simulink model "InfusionPumpPlantModel"  (R2022b)
settings: Solver=ode23t  StartTime=0.0  StopTime=10.0  MaxStep=0.001  RelTol=1e-3
undefined symbols (not defined in the file): const_Occl_Pct, reserv_str
libraries: fl_lib x44, nesl_utility x21, sh_lib x7, sdl_lib x4, ee_lib x1, simulink_extras x1, fl_ps_legacy_lib x1
settings Model: Creator=szhang  LastModifiedBy=ppatel
settings SolverCC: AlgebraicLoopSolver=TrustRegion
settings DebuggingCC: UnconnectedInputMsg=warning  UnconnectedOutputMsg=warning  UnconnectedLineMsg=warning  SFMachineParentedDataDiag=warning  ArithmeticOperatorsInVariantConditions=warning
settings ModelReferenceCC: EnableRefExpFcnMdlSchedulingChecks=on
settings SFSimCC: SimUseLocalCustomCode=off  CustomCodeUndefinedFunction=UseInterfaceOnly
settings RTWCC: RTWUseLocalCustomCode=off
settings CodeAppCC: StateflowObjectComments=on
settings SimscapeCC: SimscapeNominalValues="[{\"value\":\"10\",\"unit\":\"V\"},{\"value\":\"1\",\"unit\":\"A\"},{\"value\":\"10\",\"unit\":\"N*m\"},{\"value\":\"10\",\"unit\":\"bar\"},{\"value\":\"100\",\"unit\":\"kJ/kg\"},{\"value\":\"1\",\"unit\":\"kW\"},{\"value\":\"300\",\"unit\":\"K\"},{\"value\":\"100\",\"unit\":\"cm^3/s\"},{\"value\":\"1\",\"unit\":\"kN\"},{\"value\":\"1\",\"unit\":\"g/cm^3\"},{\"value\":\"1\",\"unit\":\"l\"},{\"value\":\"1\",\"unit\":\"cm^2\"},{\"value\":\"60\",\"unit\":\"Hz\"}]"

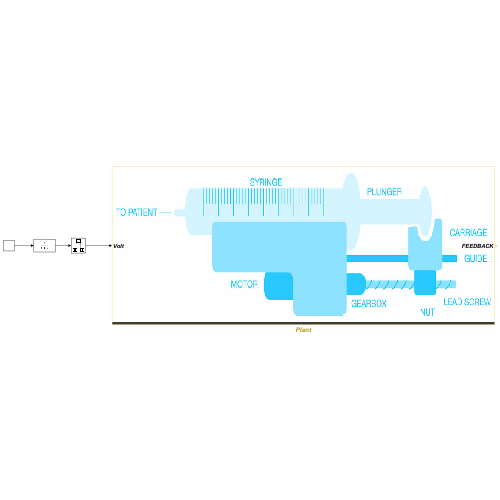
[thumbnail: Simulink's stored preview of the top-level diagram]
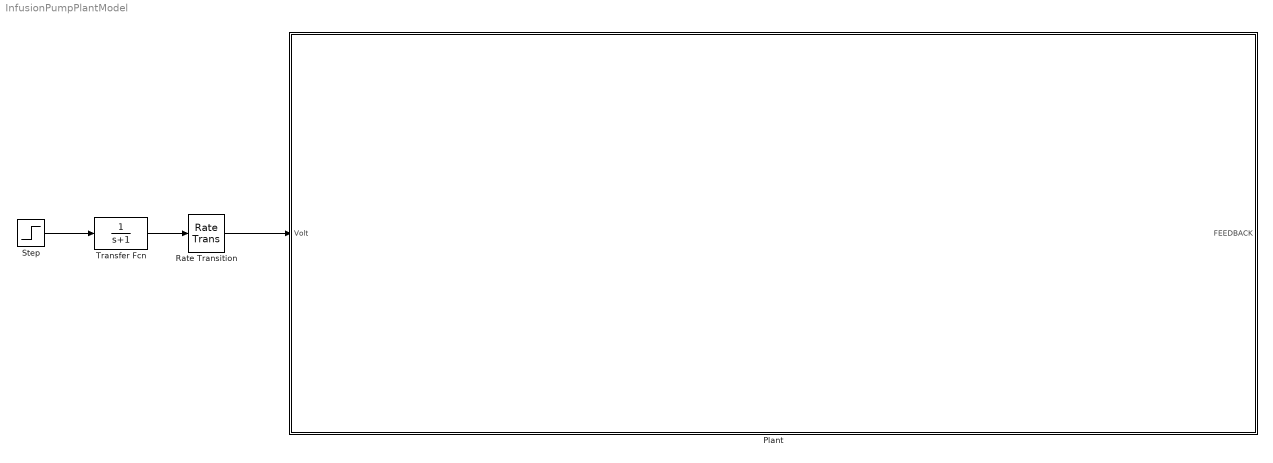
== system InfusionPumpPlantModel ==
  Plant : Subsystem
      mask Display: image('InfusionDevice.PNG');
  Rate Transition : RateTransition  OutPortSampleTime=0.001
  Step : Step  After=2.5  SampleTime=0
  Transfer Fcn : TransferFcn  Denominator=[1 1]
  wires:
  Rate Transition/1 -> Plant/1(Volt)
  Step/1 -> Transfer Fcn/1
  Transfer Fcn/1 -> Rate Transition/1

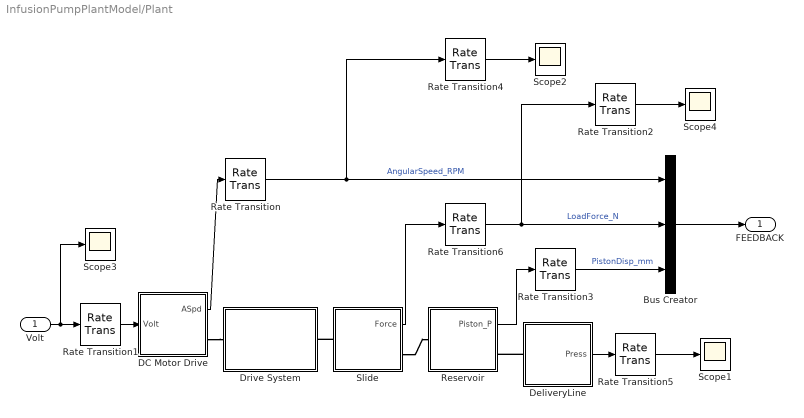
== system InfusionPumpPlantModel/Plant ==
  Volt : Inport
  Bus Creator : BusCreator  Inputs='AngularSpeed_RPM','LoadForce_N','PistonDisp_mm'  OutDataTypeStr=Bus: FEEDBACK  NonVirtualBus=on
  DC Motor Drive : Subsystem
      mask Display: image('DCMotor.PNG')
  DeliveryLine : Subsystem
      mask Display: image('DeliveryLine.PNG')
  Drive System : Subsystem
      mask Display: image('DriveSys.PNG')
  Rate Transition : RateTransition  OutPortSampleTime=0.001
  Rate Transition1 : RateTransition
  Rate Transition2 : RateTransition  OutPortSampleTime=0.01
  Rate Transition3 : RateTransition  OutPortSampleTime=0.001
  Rate Transition4 : RateTransition  OutPortSampleTime=0.01
  Rate Transition5 : RateTransition  OutPortSampleTime=0.01
  Rate Transition6 : RateTransition  OutPortSampleTime=0.001
  Reservoir : Subsystem
      mask Display: image('Reservoir.PNG')
  Scope{1..4} (4 alike) : Scope
  Slide : Subsystem
  FEEDBACK : Outport  OutDataTypeStr=Bus: FEEDBACK
  wires:
  DC Motor Drive/1(ASpd) -> Rate Transition/1
  Volt/1 -> Scope3/1, Rate Transition1/1
  Rate Transition1/1 -> DC Motor Drive/1(Volt)
  DeliveryLine/1(Press) -> Rate Transition5/1
  Rate Transition3/1 -> Bus Creator/3  "PistonDisp_mm"
  Reservoir/1(Piston_P) -> Rate Transition3/1
  Rate Transition/1 -> Rate Transition4/1, Bus Creator/1  "AngularSpeed_RPM"
  Rate Transition4/1 -> Scope2/1
  Rate Transition5/1 -> Scope1/1
  Slide/1(Force) -> Rate Transition6/1
  Rate Transition6/1 -> Rate Transition2/1, Bus Creator/2  "LoadForce_N"
  Bus Creator/1 -> FEEDBACK/1
  Rate Transition2/1 -> Scope4/1
  connections:
  Slide/RConn1 -- Reservoir/LConn1
  DC Motor Drive/RConn1 -- Drive System/LConn1
  Slide/LConn1 -- Drive System/RConn1
  DeliveryLine/LConn1 -- Reservoir/RConn1

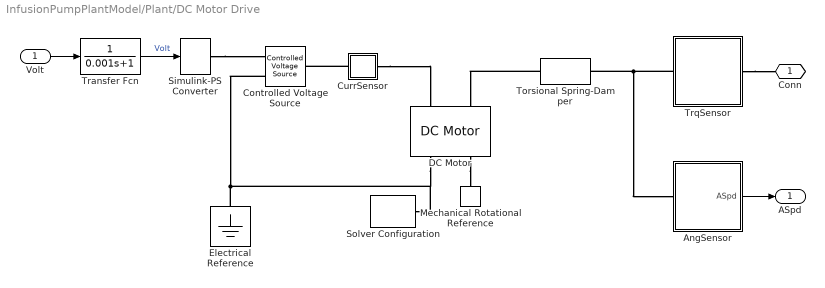
== system InfusionPumpPlantModel/Plant/DC Motor Drive ==
  Volt : Inport
  AngSensor : Subsystem
  Controlled Voltage Source : fl_lib/Electrical/Electrical Sources/Controlled Voltage Source
  CurrSensor : Subsystem
  DC Motor : ee_lib/Electromechanical/Brushed Motors/DC Motor  field_option=ee.enum.field_option.pm  Rf=100 Ohm  Lf=1 H  Laf=0.15 H  If0=0 A  parameterization=1  Ra=reserv_str.DCMotor.Resist Ohm  La=reserv_str.DCMotor.Induct H  emf_or_torque=1  Kv=reserv_str.DCMotor.BEMF V/(rad/s)  Ki=6.876e-4 N*m/A  T_stall=2.4e-4 N*m  w_max=1.91e+4 rpm  w_rated=1.5e+4 rpm  P_rated=0.08 W  V_rated=1.5 V  lam_param=1  i_noload=0 A  V_i_noload=1.5 V  J=reserv_str.DCMotor.RotorInert kg*m^2  lam=reserv_str.DCMotor.RotorDamp N*m/(rad/s)  speed0=0 rpm  enable_fault_armature=simscape.enum.onoff.off  rev_faulted=1 / 3  G_faulted_armature=1e-5 S  fault_trigger_armature=ee.enum.faults.faultTrigger.temporal  t_fault_armature=1 s  max_permissible_current_armature=inf A  t_fail_on_current_armature=1 s  enable_fault_field=simscape.enum.onoff.off  G_faulted_field=1e-5 S  fault_trigger_field=ee.enum.faults.faultTrigger.temporal  t_fault_field=1 s  max_permissible_current_field=inf A  t_fail_on_current_field=1 s  fault_action=simscape.enum.assert.action.none  alpha=3.93e-3 1/K  Tmeas=25 degC  thermal_mass=100 J/K  initial_temperature=25 degC
  Electrical Reference : fl_lib/Electrical/Electrical Elements/Electrical Reference
  Mechanical Rotational Reference : fl_lib/Mechanical/Rotational Elements/Mechanical Rotational Reference
  Simulink-PS Converter : nesl_utility/Simulink-PS Converter  PhysicalDomain=network_engine_domain  SubClassName=ps_input  LeftPortType=input  RightPortType=output  PseudoPeriodic=off  Frequencies=[]  NoiseDistribution=none  NoiseParameters=[]  Unit=1  AffineConversion=off  FilteringAndDerivatives=filter  SimscapeFilterOrder=2  InputFilterTimeConstant=0.001  UdotUserProvided=1
  Solver Configuration : nesl_utility/Solver Configuration  PhysicalDomain=network_engine_domain  SubClassName=solver  LeftPortType=input  RightPortType=generic  Tones=[]  Harmonics=[]  SimulateNoise=off  Profile=off  UseLocalSampling=off  EnableSwitchedLinearOptims=on  FrequencyDomain=off  UseCCode=off  RelTol=0.001  AbsTol=1e-06  MinStep=1e-09  ToWorkspace=off  RevertToSquareIcSolve=off  NumHomotopyIterations=100  PhasorMode=off  PhasorModeNumHarmonics=1  ConsistencySolver=NEWTON_XTOL_AFTER_FTOL  IndexReductionMethod=DerivativeReplacement  DoDC=off  ResidualTolerance=1e-09  ConsistencyTolSource=GLOBAL  ConsistencyAbsTol=0.001  ConsistencyRelTol=0.001  ConsistencyTolFactor=0.001  UseLocalSolver=off  LocalSolverChoice=NE_BACKWARD_EULER_ADVANCER  ResolveIndetEquations=on  FunctionEvalNumThread=1  LocalSolverSampleTime=0.001  DoFixedCost=off  MaxNonlinIter=3  MaxModeIter=2  ComputeImpulses=off  ImpulseIterations=2  LinearAlgebra=Sparse  LinearAlgebraNumThread=0  EquationFormulation=NE_TIME_EF  DelaysMemoryBudget=1024  AutomaticFiltering=on  FilteringTimeConstant=0.001  PartitionStorageMethod=AS_NEEDED  PartitionMemoryBudget=1024  PartitionMethod=FAST
  Torsional Spring-Damper : sdl_lib/Couplings & Drives/Torsional Spring-Damper  k=10000 N*m/rad  mu_visc=1000 N*m/(rad/s)  trq_coulomb=0 N*m  static_kinetic_ratio=1.1  w_tol=0.001 rad/s  model_hardstop=0  upper_bound=10 deg  lower_bound=-10 deg  k_endstop=1e+6 N*m/rad  D_endstop=10 N*m/(rad/s)  hardstop_model=3  transition=0.001 rad  x0=0 deg
      settings: InternalSimscapePortConfiguration="{\"Bottom\":[],\"Left\":[{\"id\":\"R\",\"label\":\"R\",\"type\":\"foundation.mechanical.rotational.rotational\"}],\"Right\":[{\"id\":\"C\",\"label\":\"C\",\"type\":\"foundation.mechanical.rotational.rotational\"}],\"Top\":[]}"
  Transfer Fcn : TransferFcn  Denominator=[0.001 1]
  TrqSensor : Subsystem
  Conn : PMIOPort  Side=Right
  ASpd : Outport
  wires:
  Volt/1 -> Transfer Fcn/1
  Transfer Fcn/1 -> Simulink-PS Converter/1  "Volt"
  AngSensor/1(ASpd) -> ASpd/1
  connections:
  Controlled Voltage Source/RConn2 -- Solver Configuration/RConn1 -- DC Motor/RConn1 -- Electrical Reference/LConn1
  DC Motor/RConn2 -- Mechanical Rotational Reference/LConn1
  Simulink-PS Converter/RConn1 -- Controlled Voltage Source/RConn1
  TrqSensor/RConn1 -- Conn/RConn1
  TrqSensor/LConn1 -- AngSensor/LConn1 -- Torsional Spring-Damper/RConn1
  CurrSensor/LConn1 -- Controlled Voltage Source/LConn1
  CurrSensor/RConn1 -- DC Motor/LConn1
  Torsional Spring-Damper/LConn1 -- DC Motor/LConn2

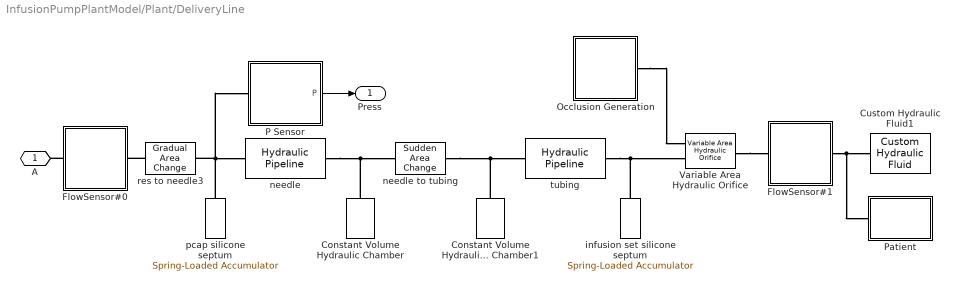
== system InfusionPumpPlantModel/Plant/DeliveryLine ==
  Constant Volume Hydraulic Chamber : fl_lib/Hydraulic/Hydraulic Elements/Constant Volume Hydraulic Chamber  ch_sp=1  wall_type=1  ch_volume=pi/4*reserv_str.Needle.Diam^2*reserv_str.Needle.Len/5 in^3  d_in=1e-2 m  length=1 m  pr_r_coef=1.2e-12 m/Pa  time_const=0.01 s  k_sh=1.4  pressure_specify=on  pressure_priority=High  pressure=reserv_str.Needle.InitP Pa  pressure_nominal_specify=off  pressure_nominal_unit=Pa  pressure_nominal_value=1  diameter_incr_specify=off  diameter_incr_priority=High  diameter_incr=0 m  diameter_incr_nominal_specify=off  diameter_incr_nominal_unit=m  diameter_incr_nominal_value=1  flow_rate_specify=off  flow_rate_priority=None  flow_rate=0.001 m^3/s  flow_rate_nominal_specify=off  flow_rate_nominal_unit=m^3/s  flow_rate_nominal_value=1
      settings: InternalSimscapePortConfiguration="{\"Bottom\":[],\"Left\":[{\"id\":\"A\",\"label\":\"\",\"type\":\"foundation.hydraulic.hydraulic\"}],\"Right\":[],\"Top\":[]}"
  Constant Volume Hydraulic Chamber1 : fl_lib/Hydraulic/Hydraulic Elements/Constant Volume Hydraulic Chamber  ch_sp=1  wall_type=1  ch_volume=pi/4*reserv_str.Tubing.Diam^2*reserv_str.Tubing.Len/5 in^3  d_in=1e-2 m  length=1 m  pr_r_coef=1.2e-12 m/Pa  time_const=0.01 s  k_sh=1.4  pressure_specify=on  pressure_priority=High  pressure=reserv_str.Needle.InitP Pa  pressure_nominal_specify=off  pressure_nominal_unit=Pa  pressure_nominal_value=1  diameter_incr_specify=off  diameter_incr_priority=High  diameter_incr=0 m  diameter_incr_nominal_specify=off  diameter_incr_nominal_unit=m  diameter_incr_nominal_value=1  flow_rate_specify=off  flow_rate_priority=None  flow_rate=0.001 m^3/s  flow_rate_nominal_specify=off  flow_rate_nominal_unit=m^3/s  flow_rate_nominal_value=1
      settings: InternalSimscapePortConfiguration="{\"Bottom\":[],\"Left\":[{\"id\":\"A\",\"label\":\"\",\"type\":\"foundation.hydraulic.hydraulic\"}],\"Right\":[],\"Top\":[]}"
  Custom Hydraulic Fluid1 : fl_lib/Hydraulic/Hydraulic Utilities/Custom Hydraulic Fluid  density=1004 kg/m^3  viscosity_kin=3.697e-6 m^2/s  bulk=2.2e9 Pa  alpha=0.0001  range_error=2
      settings: InternalSimscapePortConfiguration="{\"Bottom\":[],\"Left\":[],\"Right\":[{\"id\":\"G\",\"label\":\"\",\"type\":\"foundation.hydraulic.hydraulic\"}],\"Top\":[]}"
  FlowSensor#0 : Subsystem
  FlowSensor#1 : Subsystem
  Occlusion Generation : Subsystem
      mask Display: image('Occlusion.PNG')
  P Sensor : Subsystem
  Patient : Subsystem
  Variable Area Hydraulic Orifice : fl_lib/Hydraulic/Hydraulic Elements/Variable Area Hydraulic Orifice  C_d=1  min_area=5e-14 m^2  lam_spec=2  B_lam=0.999  Re_cr=12  q_specify=off  q_priority=High  q=1 m^3/s  q_nominal_specify=off  q_nominal_unit=m^3/s  q_nominal_value=1  p_specify=off  p_priority=High  p=0 Pa  p_nominal_specify=off  p_nominal_unit=Pa  p_nominal_value=1
      settings: InternalSimscapePortConfiguration="{\"Bottom\":[],\"Left\":[{\"id\":\"AR\",\"label\":\"AR\",\"type\":\"input\"},{\"id\":\"A\",\"label\":\"A\",\"type\":\"foundation.hydraulic.hydraulic\"}],\"Right\":[{\"id\":\"B\",\"label\":\"B\",\"type\":\"foundation.hydraulic.hydraulic\"}],\"Top\":[]}"
  infusion set silicone septum : sh_lib/Accumulators/Spring-Loaded Accumulator  capacity=reserv_str.Infu.Capacity mm^3  pr_preload=reserv_str.Infu.PreloadP Pa  pr_max=reserv_str.Infu.MaxP Pa  stiff_coeff=1e10 Pa/m^3  penetr_coeff=1e10 s*Pa/m^6  flow_rate_specify=off  flow_rate_priority=None  flow_rate=0.005 m^3/s  flow_rate_nominal_specify=off  flow_rate_nominal_unit=m^3/s  flow_rate_nominal_value=1  fluid_volume_specify=on  fluid_volume_priority=High  fluid_volume=0 m^3  fluid_volume_nominal_specify=off  fluid_volume_nominal_unit=m^3  fluid_volume_nominal_value=1  fluid_pressure_specify=off  fluid_pressure_priority=None  fluid_pressure=1.01325e+5 Pa  fluid_pressure_nominal_specify=off  fluid_pressure_nominal_unit=Pa  fluid_pressure_nominal_value=1
      settings: InternalSimscapePortConfiguration="{\"Bottom\":[],\"Left\":[],\"Right\":[{\"id\":\"A\",\"label\":\"A\",\"type\":\"foundation.hydraulic.hydraulic\"}],\"Top\":[]}"
  needle : sh_lib/Pipelines/Hydraulic Pipeline  cs_type=1  d_in=reserv_str.Needle.Diam in  area=1e-4 m^2  D_h=0.0112 m  s_factor=64  length=reserv_str.Needle.Len in  length_ad=0 in  roughness=1.5e-3 mm  Re_lam=2e3  Re_turb=4e+3  wall_type=1  pr_r_coef=2e-12 mm/Pa  time_const=0.01 s  k_sh=1.4  initial_pressure=reserv_str.Needle.InitP Pa
      settings: InternalSimscapePortConfiguration="{\"Bottom\":[],\"Left\":[{\"id\":\"A\",\"label\":\"A\",\"type\":\"foundation.hydraulic.hydraulic\"}],\"Right\":[{\"id\":\"B\",\"label\":\"B\",\"type\":\"foundation.hydraulic.hydraulic\"}],\"Top\":[]}"
  needle to tubing : sh_lib/Local Hydraulic Resistances/Sudden Area Change  mdl_type=1  small_diam=reserv_str.Needle.Diam in  large_diam=reserv_str.Tubing.Diam mm  kp_c=1  lam_spec=2  B_lam=0.999  Re_cr=110  Re_vec=[ -4e+3 -3e+3 -2e+3 -1000 -500 -200 -100 -50 -40 -30 -20 -15 -10 10 20 30 40 50 100 200 500 1000 2e+3 4e+3 5e+3 1e+4 ]  loss_coeff_vec=[ 0.25 0.3 0.65 0.9 0.65 0.75 0.9 1.15 1.35 1.65 2.3 2.8 3.1 5 2.7 1.8 1.46 1.3 0.9 0.65 0.42 0.3 0.2 0.4 0.42 0.25 ]  interp_method=2  extrap_method=2
      settings: InternalSimscapePortConfiguration="{\"Bottom\":[],\"Left\":[{\"id\":\"A\",\"label\":\"A\",\"type\":\"foundation.hydraulic.hydraulic\"}],\"Right\":[{\"id\":\"B\",\"label\":\"B\",\"type\":\"foundation.hydraulic.hydraulic\"}],\"Top\":[]}"
  pcap silicone septum : sh_lib/Accumulators/Spring-Loaded Accumulator  capacity=reserv_str.Septum.Capacity mm^3  pr_preload=reserv_str.Septum.PreloadP Pa  pr_max=reserv_str.Septum.MaxP Pa  stiff_coeff=1e10 Pa/m^3  penetr_coeff=1e10 s*Pa/m^6  flow_rate_specify=off  flow_rate_priority=None  flow_rate=0.005 m^3/s  flow_rate_nominal_specify=off  flow_rate_nominal_unit=m^3/s  flow_rate_nominal_value=1  fluid_volume_specify=on  fluid_volume_priority=High  fluid_volume=0 m^3  fluid_volume_nominal_specify=off  fluid_volume_nominal_unit=m^3  fluid_volume_nominal_value=1  fluid_pressure_specify=off  fluid_pressure_priority=None  fluid_pressure=1.01325e+5 Pa  fluid_pressure_nominal_specify=off  fluid_pressure_nominal_unit=Pa  fluid_pressure_nominal_value=1
      settings: InternalSimscapePortConfiguration="{\"Bottom\":[],\"Left\":[],\"Right\":[{\"id\":\"A\",\"label\":\"A\",\"type\":\"foundation.hydraulic.hydraulic\"}],\"Top\":[]}"
  res to needle3 : sh_lib/Local Hydraulic Resistances/Gradual Area Change  mdl_type=1  small_diam=reserv_str.Needle.Diam in  large_diam=reserv_str.Resvor.InDiam in  angle=reserv_str.Needle.Ang deg  kp_c=1  lam_spec=2  B_lam=0.999  Re_cr=350  Re_vec=[ -1e+4 -5e+3 -4e+3 -2e+3 -1000 -500 -200 -100 -50 -40 -30 -20 -10 10 20 30 40 50 100 200 500 1000 2e+3 4e+3 5e+3 1e+4 ]  loss_coeff_vec=[ 0.05 0.05 0.06 0.09 0.15 0.26 0.4 0.61 0.91 1.12 1.48 2.23 4.4 4 1.9 1.26 0.9399999999999999 0.76 0.52 0.48 0.42 0.36 0.24 0.4 0.42 0.35 ]  interp_method=2  extrap_method=2
      settings: InternalSimscapePortConfiguration="{\"Bottom\":[],\"Left\":[{\"id\":\"A\",\"label\":\"A\",\"type\":\"foundation.hydraulic.hydraulic\"}],\"Right\":[{\"id\":\"B\",\"label\":\"B\",\"type\":\"foundation.hydraulic.hydraulic\"}],\"Top\":[]}"
  tubing : sh_lib/Pipelines/Hydraulic Pipeline  cs_type=1  d_in=reserv_str.Tubing.Diam mm  area=1e-4 m^2  D_h=0.0112 m  s_factor=64  length=reserv_str.Tubing.Len*2.54 cm  length_ad=0 cm  roughness=1.5e-3 mm  Re_lam=2000  Re_turb=4000  wall_type=2  pr_r_coef=reserv_str.Tubing.Compliance m/Pa  time_const=0.01 s  k_sh=1.4  initial_pressure=reserv_str.Tubing.InitP Pa
      settings: InternalSimscapePortConfiguration="{\"Bottom\":[],\"Left\":[{\"id\":\"A\",\"label\":\"A\",\"type\":\"foundation.hydraulic.hydraulic\"}],\"Right\":[{\"id\":\"B\",\"label\":\"B\",\"type\":\"foundation.hydraulic.hydraulic\"}],\"Top\":[]}"
  A : PMIOPort  Side=Left
  Press : Outport
  wires:
  P Sensor/1(P) -> Press/1
  connections:
  needle/RConn1 -- Constant Volume Hydraulic Chamber/LConn1 -- needle to tubing/LConn1
  res to needle3/RConn1 -- FlowSensor#0/RConn1
  pcap silicone septum/RConn1 -- res to needle3/LConn1 -- P Sensor/LConn1 -- needle/LConn1
  needle to tubing/RConn1 -- Constant Volume Hydraulic Chamber1/LConn1 -- tubing/LConn1
  FlowSensor#1/RConn1 -- Patient/LConn1 -- Custom Hydraulic Fluid1/RConn1
  FlowSensor#0/LConn1 -- A/RConn1
  Variable Area Hydraulic Orifice/RConn1 -- FlowSensor#1/LConn1
  tubing/RConn1 -- infusion set silicone septum/RConn1 -- Variable Area Hydraulic Orifice/LConn2
  Occlusion Generation/RConn1 -- Variable Area Hydraulic Orifice/LConn1

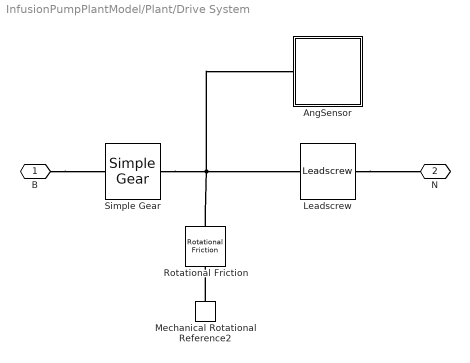
== system InfusionPumpPlantModel/Plant/Drive System ==
  AngSensor : Subsystem
  Leadscrew : sdl_lib/Gears/Rotational- Translational/Leadscrew  Lead=reserv_str.DriveSys.ScrewLead in  helix_type=2  friction_model=2  friction_parameterization=1  lambda=reserv_str.DriveSys.LeadAng deg  alpha=reserv_str.DriveSys.AcmeHalfAng deg  fr_coeff=reserv_str.DriveSys.FricCoeff  eff_sn=0.39  eff_ns=-0.5  temperature_TLU=[ 280 300 320 ] K  efficiency_sn_TLU=[ 0.75 0.7 0.65 ]  efficiency_ns_TLU=[ 0.5 0.45 0.4 ]  pwr_thr=reserv_str.DriveSys.FricCoeff W  mu_visc=reserv_str.DriveSys.DepdFricCoeff N*m/(rad/s)  thermal_mass=50 J/K  temperature_specify=off  temperature_priority=High  temperature=300 K  temperature_nominal_specify=off  temperature_nominal_unit=K  temperature_nominal_value=1
      settings: InternalSimscapePortConfiguration="{\"Bottom\":[],\"Left\":[{\"id\":\"S\",\"label\":\"S\",\"type\":\"foundation.mechanical.rotational.rotational\"}],\"Right\":[{\"id\":\"N\",\"label\":\"N\",\"type\":\"foundation.mechanical.translational.translational\"}],\"Top\":[]}"
  Mechanical Rotational Reference2 : fl_lib/Mechanical/Rotational Elements/Mechanical Rotational Reference
  Rotational Friction : fl_lib/Mechanical/Rotational Elements/Rotational Friction  brkwy_trq=10 mm*N  brkwy_vel=0.060623 rad/s  Col_trq=8 mm*N  visc_coef=0.001 N*m/(rad/s)  w_specify=off  w_priority=High  w=0 rad/s  w_nominal_specify=off  w_nominal_unit=rad/s  w_nominal_value=1  t_specify=off  t_priority=High  t=0 N*m  t_nominal_specify=off  t_nominal_unit=N*m  t_nominal_value=1
  Simple Gear : sdl_lib/Gears/Simple Gear  ratio=reserv_str.DriveSys.GearRatio  rotation_direction=3-2*(2)  friction_model=2  T_noload=0.1 N*m  T_nom=5 N*m  efficiency_nom=0.8  efficiency=reserv_str.DriveSys.GearEff  temperature_TLU=[ 280 300 320 ] K  load_TLU=[ 1 5 10 ] N*m  efficiency_TLU=[ 0.95 0.9 0.85 ]  efficiency_TLU2=[ 0.85 0.8 0.75; 0.95 0.9 0.85; 0.85 0.8 0.7 ]  w_thr=0.01 rad/s  pwr_thr=0.001 W  backlash_model=sdl.enum.backlashModel.Off  backlash_distance=1e-3 mm  x0=0 mm  r_base=0.1 m  hardstop_model=simscape.enum.hardstop.smooth  transition=1e-4 mm  backlash_stiffness=1e7 N/m  backlash_damping=1e6 N*s/m  e=0  v_tol=0.001 m/s  mu_visc=[0 0] N*m/(rad/s)  enable_faults=simscape.enum.onoff.off  efficiency_fault=0.05  external_fault=simscape.enum.onoff.off  temporal_fault=simscape.enum.onoff.off  fault_time=5 s  fault_angles=pi / 12 rad  report_fault=simscape.enum.assert.action.none  thermal_mass=50 J/K  temperature_specify=off  temperature_priority=High  temperature=300 K  temperature_nominal_specify=off  temperature_nominal_unit=K  temperature_nominal_value=1  x_backlash_specify=off  x_backlash_priority=None  x_backlash=0 mm  x_backlash_nominal_specify=off  x_backlash_nominal_unit=mm  x_backlash_nominal_value=1  f_hardstop_specify=off  f_hardstop_priority=None  f_hardstop=0 N  f_hardstop_nominal_specify=off  f_hardstop_nominal_unit=N  f_hardstop_nominal_value=1  v_backlash_specify=off  v_backlash_priority=None  v_backlash=0 m/s  v_backlash_nominal_specify=off  v_backlash_nominal_unit=m/s  v_backlash_nominal_value=1
  B : PMIOPort  Side=Left
  N : PMIOPort  Port=2  Side=Right
  connections:
  B/RConn1 -- Simple Gear/LConn1
  Mechanical Rotational Reference2/LConn1 -- Rotational Friction/LConn1
  Simple Gear/RConn1 -- Leadscrew/LConn1 -- Rotational Friction/RConn1 -- AngSensor/LConn1
  Leadscrew/RConn1 -- N/RConn1

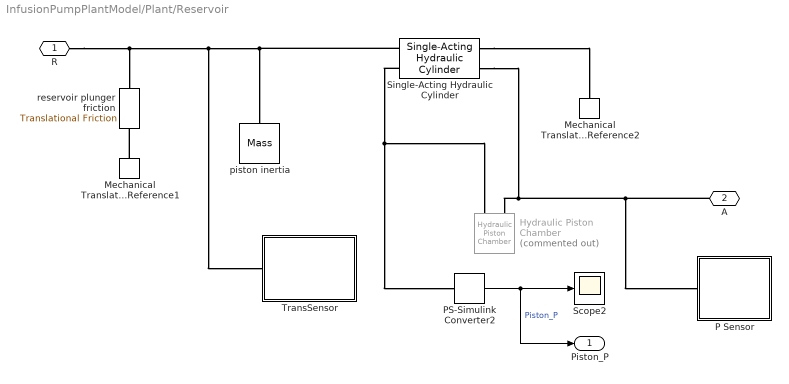
== system InfusionPumpPlantModel/Plant/Reservoir ==
  Hydraulic Piston Chamber : fl_lib/Hydraulic/Hydraulic Elements/Hydraulic Piston Chamber  Commented=on  area=reserv_str.Resvor.Area m^2  init_pos=0 mm  or=2  V_dead=1e-4 m^3  k_sh=1.4  pressure_specify=on  pressure_priority=High  pressure=reserv_str.Resvor.InitP Pa  pressure_nominal_specify=off  pressure_nominal_unit=Pa  pressure_nominal_value=1  chamber_flow_rate_specify=off  chamber_flow_rate_priority=None  chamber_flow_rate=0.001 m^3/s  chamber_flow_rate_nominal_specify=off  chamber_flow_rate_nominal_unit=m^3/s  chamber_flow_rate_nominal_value=1
      settings: InternalSimscapePortConfiguration="{\"Bottom\":[],\"Left\":[{\"id\":\"P\",\"label\":\"P\",\"type\":\"input\"},{\"id\":\"A\",\"label\":\"A\",\"type\":\"foundation.hydraulic.hydraulic\"}],\"Right\":[],\"Top\":[]}"
  Mechanical Translational Reference1 : fl_lib/Mechanical/Translational Elements/Mechanical Translational Reference
  Mechanical Translational Reference2 : fl_lib/Mechanical/Translational Elements/Mechanical Translational Reference
  P Sensor : Subsystem
  PS-Simulink Converter2 : nesl_utility/PS-Simulink Converter  PhysicalDomain=network_engine_domain  SubClassName=ps_output  LeftPortType=input  RightPortType=output  PseudoPeriodic=off  Frequencies=[]  VectorFormat=1-D array  Unit=mm  AffineConversion=off
  Scope2 : Scope
  Single-Acting Hydraulic Cylinder : sh_lib/Hydraulic Cylinders/Single-Acting Hydraulic Cylinder  area=reserv_str.Resvor.Area mm^2  stroke=reserv_str.Resvor.Len mm  displacement_spec=foundation.enum.DisplacementSpec.Calculate  init_pos=reserv_str.Resvor.Len mm  dead_vol=1e-4 m^3  init_pressure=reserv_str.Resvor.InitP Pa  k_sh=1.4  stiff=1e6 N/m  D=1500 N/(m/s)  hardstop_model=3  transition=0.1 mm  or=2
      settings: InternalSimscapePortConfiguration="{\"Bottom\":[],\"Left\":[{\"id\":\"C\",\"label\":\"C\",\"type\":\"foundation.mechanical.translational.translational\"},{\"id\":\"A\",\"label\":\"A\",\"type\":\"foundation.hydraulic.hydraulic\"}],\"Right\":[{\"id\":\"R\",\"label\":\"R\",\"type\":\"foundation.mechanical.translational.translational\"},{\"id\":\"P\",\"label\":\"p\",\"type\":\"output\"}],\"Top\":[]}"
  TransSensor : Subsystem
  piston inertia : fl_lib/Mechanical/Translational Elements/Mass  mass=reserv_str.Resvor.PistonMass*10 kg  num_ports=foundation.enum.numPorts2.one  v_specify=on  v_priority=High  v=0 m/s  v_nominal_specify=off  v_nominal_unit=m/s  v_nominal_value=1  f_specify=off  f_priority=High  f=0 N  f_nominal_specify=off  f_nominal_unit=N  f_nominal_value=1
  reservoir plunger friction : fl_lib/Mechanical/Translational Elements/Translational Friction  brkwy_frc=reserv_str.Resvor.Brkaway N  brkwy_vel=exp(-( (reserv_str.Resvor.LinVelThresh) * 1 * (reserv_str.Resvor.TransApproxCoeff) * 1 + 1/2) ) * ( (reserv_str.Resvor.LinVelThresh) * 1 / 2 + 1 / ( (reserv_str.Resvor.TransApproxCoeff) * 1) ) m/s  Col_frc=reserv_str.Resvor.Coulomb N  visc_coef=reserv_str.Resvor.ViscFric N/(m/s)  v_specify=off  v_priority=High  v=0 m/s  v_nominal_specify=off  v_nominal_unit=m/s  v_nominal_value=1  f_specify=off  f_priority=High  f=0 N  f_nominal_specify=off  f_nominal_unit=N  f_nominal_value=1
      settings: InternalSimscapePortConfiguration="{\"Bottom\":[],\"Left\":[{\"id\":\"R\",\"label\":\"R\",\"type\":\"foundation.mechanical.translational.translational\"}],\"Right\":[{\"id\":\"C\",\"label\":\"C\",\"type\":\"foundation.mechanical.translational.translational\"}],\"Top\":[]}"
  R : PMIOPort  Side=Left
  A : PMIOPort  Port=2  Side=Right
  Piston_P : Outport
  wires:
  PS-Simulink Converter2/1 -> Piston_P/1, Scope2/1  "Piston_P"
  connections:
  Mechanical Translational Reference1/LConn1 -- reservoir plunger friction/RConn1
  Single-Acting Hydraulic Cylinder/LConn1 -- Mechanical Translational Reference2/LConn1
  Single-Acting Hydraulic Cylinder/RConn2 -- PS-Simulink Converter2/LConn1 -- Hydraulic Piston Chamber/LConn1
  Hydraulic Piston Chamber/LConn2 -- P Sensor/LConn1 -- A/RConn1 -- Single-Acting Hydraulic Cylinder/LConn2
  Single-Acting Hydraulic Cylinder/RConn1 -- TransSensor/LConn1 -- R/RConn1 -- reservoir plunger friction/LConn1 -- piston inertia/LConn1

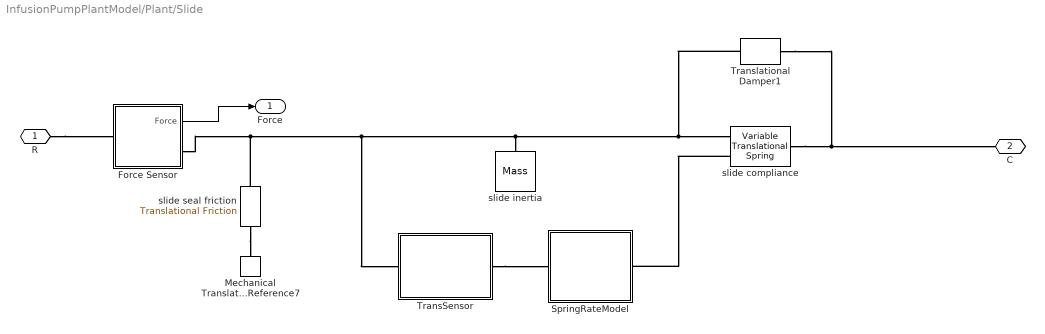
== system InfusionPumpPlantModel/Plant/Slide ==
  Force Sensor : Subsystem
  Mechanical Translational Reference7 : fl_lib/Mechanical/Translational Elements/Mechanical Translational Reference
  SpringRateModel : Subsystem  mask{E=reserv_str.Slide.EMod, A=reserv_str.Slide.CrosA, InitL=reserv_str.Slide.InitL}
      mask prompts: E "Young's Modulus (Pa)"; A "Cross-sectional Area (m^2)"; InitL "Initial Length (m)"
  TransSensor : Subsystem
  Translational Damper1 : fl_lib/Mechanical/Translational Elements/Translational Damper  D=10000 N/(m/s)  v_specify=off  v_priority=None  v=0 m/s  v_nominal_specify=off  v_nominal_unit=m/s  v_nominal_value=1  f_specify=off  f_priority=None  f=0 N  f_nominal_specify=off  f_nominal_unit=N  f_nominal_value=1
  slide compliance : sdl_lib/Couplings & Drives/Springs & Dampers/Variable Translational Spring  Kmin=reserv_str.Slide.MinSprRate N/m  x_specify=on  x_priority=High  x=reserv_str.Slide.InitDeform mm  x_nominal_specify=off  x_nominal_unit=m  x_nominal_value=1
      settings: InternalSimscapePortConfiguration="{\"Bottom\":[],\"Left\":[{\"id\":\"K\",\"label\":\"K\",\"type\":\"input\"},{\"id\":\"R\",\"label\":\"R\",\"type\":\"foundation.mechanical.translational.translational\"}],\"Right\":[{\"id\":\"C\",\"label\":\"C\",\"type\":\"foundation.mechanical.translational.translational\"}],\"Top\":[]}"
  slide inertia : fl_lib/Mechanical/Translational Elements/Mass  mass=reserv_str.Slide.Mass kg  num_ports=foundation.enum.numPorts2.one  v_specify=on  v_priority=High  v=0 m/s  v_nominal_specify=off  v_nominal_unit=m/s  v_nominal_value=1  f_specify=off  f_priority=High  f=0 N  f_nominal_specify=off  f_nominal_unit=N  f_nominal_value=1
  slide seal friction : fl_lib/Mechanical/Translational Elements/Translational Friction  brkwy_frc=reserv_str.Slide.Brkaway N  brkwy_vel=exp(-( (reserv_str.Slide.LinVelThresh) * 1 * (reserv_str.Slide.TransApproxCoeff) * 1 + 1/2) ) * ( (reserv_str.Slide.LinVelThresh) * 1 / 2 + 1 / ( (reserv_str.Slide.TransApproxCoeff) * 1) ) m/s  Col_frc=reserv_str.Slide.Coulomb N  visc_coef=reserv_str.Slide.ViscFric N/(m/s)  v_specify=off  v_priority=High  v=0 m/s  v_nominal_specify=off  v_nominal_unit=m/s  v_nominal_value=1  f_specify=off  f_priority=High  f=0 N  f_nominal_specify=off  f_nominal_unit=N  f_nominal_value=1
      settings: InternalSimscapePortConfiguration="{\"Bottom\":[],\"Left\":[{\"id\":\"R\",\"label\":\"R\",\"type\":\"foundation.mechanical.translational.translational\"}],\"Right\":[{\"id\":\"C\",\"label\":\"C\",\"type\":\"foundation.mechanical.translational.translational\"}],\"Top\":[]}"
  R : PMIOPort  Side=Left
  C : PMIOPort  Port=2  Side=Right
  Force : Outport
  wires:
  Force Sensor/1(Force) -> Force/1
  connections:
  Force Sensor/RConn1 -- slide seal friction/LConn1 -- TransSensor/LConn1 -- Translational Damper1/LConn1 -- slide compliance/LConn2 -- slide inertia/LConn1
  slide compliance/RConn1 -- Translational Damper1/RConn1 -- C/RConn1
  slide compliance/LConn1 -- SpringRateModel/RConn1
  TransSensor/RConn1 -- SpringRateModel/LConn1
  slide seal friction/RConn1 -- Mechanical Translational Reference7/LConn1
  R/RConn1 -- Force Sensor/LConn1

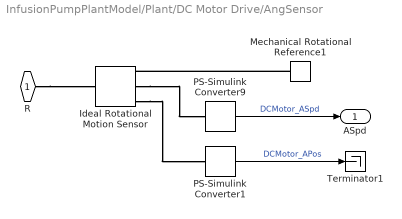
== system InfusionPumpPlantModel/Plant/DC Motor Drive/AngSensor ==
  Ideal Rotational Motion Sensor : fl_lib/Mechanical/Mechanical Sensors/Ideal Rotational Motion Sensor  reference=foundation.enum.MeasurementReference.difference  acceleration_port=false  velocity_port=true  position_port=true  wrap_angle=false  offset=0 rad
  Mechanical Rotational Reference1 : fl_lib/Mechanical/Rotational Elements/Mechanical Rotational Reference
  PS-Simulink Converter1 : nesl_utility/PS-Simulink Converter  PhysicalDomain=network_engine_domain  SubClassName=ps_output  LeftPortType=input  RightPortType=output  PseudoPeriodic=off  Frequencies=[]  VectorFormat=1-D array  Unit=rad  AffineConversion=off
  PS-Simulink Converter9 : nesl_utility/PS-Simulink Converter  PhysicalDomain=network_engine_domain  SubClassName=ps_output  LeftPortType=input  RightPortType=output  PseudoPeriodic=off  Frequencies=[]  VectorFormat=1-D array  Unit=rpm  AffineConversion=off
  Terminator1 : Terminator
  R : PMIOPort  Side=Left
  ASpd : Outport
  wires:
  PS-Simulink Converter1/1 -> Terminator1/1  "DCMotor_APos"
  PS-Simulink Converter9/1 -> ASpd/1  "DCMotor_ASpd"
  connections:
  Mechanical Rotational Reference1/LConn1 -- Ideal Rotational Motion Sensor/RConn1
  Ideal Rotational Motion Sensor/RConn2 -- PS-Simulink Converter9/LConn1
  Ideal Rotational Motion Sensor/RConn3 -- PS-Simulink Converter1/LConn1
  R/RConn1 -- Ideal Rotational Motion Sensor/LConn1

== system InfusionPumpPlantModel/Plant/DC Motor Drive/CurrSensor ==
  Current Sensor1 : fl_lib/Electrical/Electrical Sensors/Current Sensor
  PS-Simulink Converter11 : nesl_utility/PS-Simulink Converter  PhysicalDomain=network_engine_domain  SubClassName=ps_output  LeftPortType=input  RightPortType=output  PseudoPeriodic=off  Frequencies=[]  VectorFormat=1-D array  Unit=A  AffineConversion=off
  Terminator : Terminator
  + : PMIOPort  Side=Left
  - : PMIOPort  Port=2  Side=Right
  wires:
  PS-Simulink Converter11/1 -> Terminator/1
  connections:
  Current Sensor1/RConn2 -- -/RConn1
  Current Sensor1/LConn1 -- +/RConn1
  Current Sensor1/RConn1 -- PS-Simulink Converter11/LConn1

== system InfusionPumpPlantModel/Plant/DC Motor Drive/TrqSensor ==
  Ideal Torque Sensor1 : fl_lib/Mechanical/Mechanical Sensors/Ideal Torque Sensor
  PS-Simulink Converter10 : nesl_utility/PS-Simulink Converter  PhysicalDomain=network_engine_domain  SubClassName=ps_output  LeftPortType=input  RightPortType=output  PseudoPeriodic=off  Frequencies=[]  VectorFormat=1-D array  Unit=N*m  AffineConversion=off
  Terminator : Terminator
  C : PMIOPort  Side=Right
  R : PMIOPort  Port=2  Side=Left
  wires:
  PS-Simulink Converter10/1 -> Terminator/1  "DCMotor_Torque"
  connections:
  Ideal Torque Sensor1/RConn1 -- C/RConn1
  Ideal Torque Sensor1/RConn2 -- PS-Simulink Converter10/LConn1
  Ideal Torque Sensor1/LConn1 -- R/RConn1

== system InfusionPumpPlantModel/Plant/DeliveryLine/FlowSensor#0 ==
  Hydraulic Flow Rate Sensor : fl_lib/Hydraulic/Hydraulic Sensors/Hydraulic Flow Rate Sensor
  PS-Simulink Converter : nesl_utility/PS-Simulink Converter  PhysicalDomain=network_engine_domain  SubClassName=ps_output  LeftPortType=input  RightPortType=output  PseudoPeriodic=off  Frequencies=[]  VectorFormat=1-D array  Unit=mm^3/min  AffineConversion=off
  Saturation : Saturate  UpperLimit=inf  LowerLimit=0
  Scope : Scope
  A : PMIOPort  Side=Left
  B : PMIOPort  Port=2  Side=Right
  wires:
  PS-Simulink Converter/1 -> Saturation/1
  Saturation/1 -> Scope/1
  connections:
  Hydraulic Flow Rate Sensor/RConn1 -- PS-Simulink Converter/LConn1
  Hydraulic Flow Rate Sensor/RConn2 -- B/RConn1
  A/RConn1 -- Hydraulic Flow Rate Sensor/LConn1

== system InfusionPumpPlantModel/Plant/DeliveryLine/FlowSensor#1 ==
  Hydraulic Flow Rate Sensor : fl_lib/Hydraulic/Hydraulic Sensors/Hydraulic Flow Rate Sensor
  PS-Simulink Converter : nesl_utility/PS-Simulink Converter  PhysicalDomain=network_engine_domain  SubClassName=ps_output  LeftPortType=input  RightPortType=output  PseudoPeriodic=off  Frequencies=[]  VectorFormat=1-D array  Unit=mm^3/min  AffineConversion=off
  Saturation : Saturate  Commented=through  UpperLimit=5000  LowerLimit=0
  Scope : Scope
  A : PMIOPort  Side=Left
  B : PMIOPort  Port=2  Side=Right
  wires:
  PS-Simulink Converter/1 -> Saturation/1
  Saturation/1 -> Scope/1
  connections:
  A/RConn1 -- Hydraulic Flow Rate Sensor/LConn1
  Hydraulic Flow Rate Sensor/RConn2 -- B/RConn1
  Hydraulic Flow Rate Sensor/RConn1 -- PS-Simulink Converter/LConn1

== system InfusionPumpPlantModel/Plant/DeliveryLine/Occlusion Generation ==
  Scope : Scope
  Simulink-PS Converter1 : nesl_utility/Simulink-PS Converter  PhysicalDomain=network_engine_domain  SubClassName=ps_input  LeftPortType=input  RightPortType=output  PseudoPeriodic=off  Frequencies=[]  NoiseDistribution=none  NoiseParameters=[]  Unit=1  AffineConversion=off  FilteringAndDerivatives=zero  SimscapeFilterOrder=1  InputFilterTimeConstant=0.001  UdotUserProvided=1
  Step1 : Step  Time=reserv_str.Occl.Time  Before=reserv_str.Tubing.Area  After=reserv_str.Tubing.Area*(1-const_Occl_Pct)  SampleTime=0
  Transfer Fcn (with initial outputs) : simulink_extras/Additional Linear/Transfer Fcn (with initial outputs)  N=[1]  D="[1  1]"  Y0=reserv_str.Tubing.Area  U0=0
  Conn1 : PMIOPort  Side=Right
  wires:
  Step1/1 -> Transfer Fcn (with initial outputs)/1
  Transfer Fcn (with initial outputs)/1 -> Scope/1, Simulink-PS Converter1/1
  connections:
  Simulink-PS Converter1/RConn1 -- Conn1/RConn1

== system InfusionPumpPlantModel/Plant/DeliveryLine/P Sensor ==
  Hydraulic Pressure Sensor : fl_lib/Hydraulic/Hydraulic Sensors/Hydraulic Pressure Sensor
  Hydraulic Reference : fl_lib/Hydraulic/Hydraulic Elements/Hydraulic Reference
  PS-Simulink Converter : nesl_utility/PS-Simulink Converter  PhysicalDomain=network_engine_domain  SubClassName=ps_output  LeftPortType=input  RightPortType=output  PseudoPeriodic=off  Frequencies=[]  VectorFormat=1-D array  Unit=1  AffineConversion=off
  A : PMIOPort  Side=Left
  P : Outport
  wires:
  PS-Simulink Converter/1 -> P/1  "Press2"
  connections:
  Hydraulic Pressure Sensor/RConn1 -- Hydraulic Reference/LConn1
  Hydraulic Pressure Sensor/RConn2 -- PS-Simulink Converter/LConn1
  A/RConn1 -- Hydraulic Pressure Sensor/LConn1

== system InfusionPumpPlantModel/Plant/DeliveryLine/Patient ==
  Hydraulic Pressure Source : fl_lib/Hydraulic/Hydraulic Sources/Hydraulic Pressure Source
      settings: InternalSimscapePortConfiguration="{\"Bottom\":[],\"Left\":[{\"id\":\"P\",\"label\":\"P\",\"type\":\"foundation.hydraulic.hydraulic\"}],\"Right\":[{\"id\":\"S\",\"label\":\"S\",\"type\":\"input\"},{\"id\":\"T\",\"label\":\"T\",\"type\":\"foundation.hydraulic.hydraulic\"}],\"Top\":[]}"
  Hydraulic Reference1 : fl_lib/Hydraulic/Hydraulic Elements/Hydraulic Reference
  PS Constant : fl_lib/Physical Signals/Sources/PS Constant  constant=101325
  P : PMIOPort  Side=Left
  connections:
  P/RConn1 -- Hydraulic Pressure Source/LConn1
  Hydraulic Reference1/LConn1 -- Hydraulic Pressure Source/RConn2
  PS Constant/RConn1 -- Hydraulic Pressure Source/RConn1

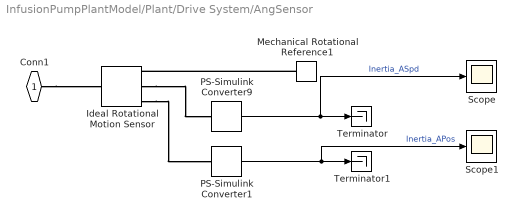
== system InfusionPumpPlantModel/Plant/Drive System/AngSensor ==
  Ideal Rotational Motion Sensor : fl_lib/Mechanical/Mechanical Sensors/Ideal Rotational Motion Sensor  reference=foundation.enum.MeasurementReference.difference  acceleration_port=false  velocity_port=true  position_port=true  wrap_angle=false  offset=0 rad
  Mechanical Rotational Reference1 : fl_lib/Mechanical/Rotational Elements/Mechanical Rotational Reference
  PS-Simulink Converter1 : nesl_utility/PS-Simulink Converter  PhysicalDomain=network_engine_domain  SubClassName=ps_output  LeftPortType=input  RightPortType=output  PseudoPeriodic=off  Frequencies=[]  VectorFormat=1-D array  Unit=rad  AffineConversion=off
  PS-Simulink Converter9 : nesl_utility/PS-Simulink Converter  PhysicalDomain=network_engine_domain  SubClassName=ps_output  LeftPortType=input  RightPortType=output  PseudoPeriodic=off  Frequencies=[]  VectorFormat=1-D array  Unit=rpm  AffineConversion=off
  Scope : Scope
  Scope1 : Scope
  Terminator : Terminator
  Terminator1 : Terminator
  Conn1 : PMIOPort  Side=Left
  wires:
  PS-Simulink Converter1/1 -> Scope1/1, Terminator1/1  "Inertia_APos"
  PS-Simulink Converter9/1 -> Scope/1, Terminator/1  "Inertia_ASpd"
  connections:
  Mechanical Rotational Reference1/LConn1 -- Ideal Rotational Motion Sensor/RConn1
  Ideal Rotational Motion Sensor/RConn2 -- PS-Simulink Converter9/LConn1
  Ideal Rotational Motion Sensor/RConn3 -- PS-Simulink Converter1/LConn1
  Conn1/RConn1 -- Ideal Rotational Motion Sensor/LConn1

== system InfusionPumpPlantModel/Plant/Reservoir/P Sensor ==
  Hydraulic Pressure Sensor : fl_lib/Hydraulic/Hydraulic Sensors/Hydraulic Pressure Sensor
  Hydraulic Reference : fl_lib/Hydraulic/Hydraulic Elements/Hydraulic Reference
  PS-Simulink Converter : nesl_utility/PS-Simulink Converter  PhysicalDomain=network_engine_domain  SubClassName=ps_output  LeftPortType=input  RightPortType=output  PseudoPeriodic=off  Frequencies=[]  VectorFormat=1-D array  Unit=1  AffineConversion=off
  Scope1 : Scope
  A : PMIOPort  Side=Left
  wires:
  PS-Simulink Converter/1 -> Scope1/1  "Press1"
  connections:
  Hydraulic Pressure Sensor/RConn1 -- Hydraulic Reference/LConn1
  Hydraulic Pressure Sensor/RConn2 -- PS-Simulink Converter/LConn1
  A/RConn1 -- Hydraulic Pressure Sensor/LConn1

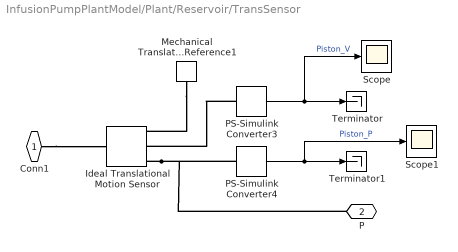
== system InfusionPumpPlantModel/Plant/Reservoir/TransSensor ==
  Ideal Translational Motion Sensor : fl_lib/Mechanical/Mechanical Sensors/Ideal Translational Motion Sensor  reference=foundation.enum.MeasurementReference.difference  acceleration_port=false  velocity_port=true  position_port=true  offset=0 m
  Mechanical Translational Reference1 : fl_lib/Mechanical/Translational Elements/Mechanical Translational Reference
  PS-Simulink Converter3 : nesl_utility/PS-Simulink Converter  PhysicalDomain=network_engine_domain  SubClassName=ps_output  LeftPortType=input  RightPortType=output  PseudoPeriodic=off  Frequencies=[]  VectorFormat=1-D array  Unit=mm/min  AffineConversion=off
  PS-Simulink Converter4 : nesl_utility/PS-Simulink Converter  PhysicalDomain=network_engine_domain  SubClassName=ps_output  LeftPortType=input  RightPortType=output  PseudoPeriodic=off  Frequencies=[]  VectorFormat=1-D array  Unit=mm  AffineConversion=off
  Scope : Scope
  Scope1 : Scope
  Terminator : Terminator
  Terminator1 : Terminator
  Conn1 : PMIOPort  Side=Left
  P : PMIOPort  Port=2  Side=Right
  wires:
  PS-Simulink Converter4/1 -> Scope1/1, Terminator1/1  "Piston_P"
  PS-Simulink Converter3/1 -> Scope/1, Terminator/1  "Piston_V"
  connections:
  Conn1/RConn1 -- Ideal Translational Motion Sensor/LConn1
  Ideal Translational Motion Sensor/RConn3 -- P/RConn1 -- PS-Simulink Converter4/LConn1
  PS-Simulink Converter3/LConn1 -- Ideal Translational Motion Sensor/RConn2
  Mechanical Translational Reference1/LConn1 -- Ideal Translational Motion Sensor/RConn1

== system InfusionPumpPlantModel/Plant/Slide/Force Sensor ==
  Ideal Force Sensor1 : fl_lib/Mechanical/Mechanical Sensors/Ideal Force Sensor
  PS-Simulink Converter15 : nesl_utility/PS-Simulink Converter  PhysicalDomain=network_engine_domain  SubClassName=ps_output  LeftPortType=input  RightPortType=output  PseudoPeriodic=off  Frequencies=[]  VectorFormat=1-D array  Unit=N  AffineConversion=off
  Terminator : Terminator
  C : PMIOPort  Side=Right
  R : PMIOPort  Port=2  Side=Left
  Force : Outport
  wires:
  PS-Simulink Converter15/1 -> Force/1, Terminator/1  "Slide_Force"
  connections:
  Ideal Force Sensor1/LConn1 -- R/RConn1
  PS-Simulink Converter15/LConn1 -- Ideal Force Sensor1/RConn2
  C/RConn1 -- Ideal Force Sensor1/RConn1

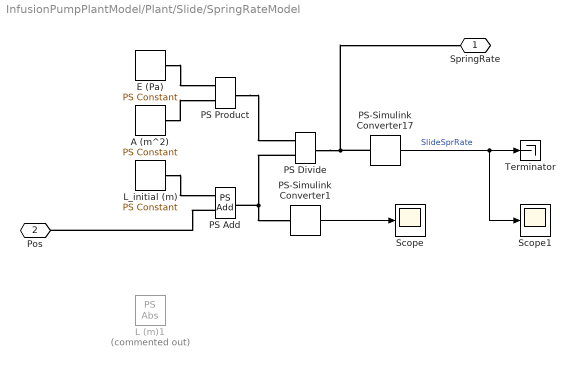
== system InfusionPumpPlantModel/Plant/Slide/SpringRateModel ==
  A (m^2) : fl_lib/Physical Signals/Sources/PS Constant  constant=A m^2
  E (Pa) : fl_lib/Physical Signals/Sources/PS Constant  constant=E Pa
  L (m)1 : fl_ps_legacy_lib/Legacy Physical Signals/Nonlinear Operators/PS Abs  Commented=on
      settings: InternalSimscapePortConfiguration="{\"Bottom\":[],\"Left\":[{\"id\":\"I\",\"label\":\"\",\"type\":\"input\"}],\"Right\":[{\"id\":\"O\",\"label\":\"\",\"type\":\"output\"}],\"Top\":[]}"
  L_initial (m) : fl_lib/Physical Signals/Sources/PS Constant  constant=InitL m
  PS Add : fl_lib/Physical Signals/Functions/PS Add
      settings: LibrarySourceBlock=|
      | fl_ps_legacy_lib/Legacy Physical
      | Signals/Functions/PS Add
  PS Divide : fl_lib/Physical Signals/Functions/PS Divide
      settings: LibrarySourceBlock=|
      | fl_ps_legacy_lib/Legacy Physical
      | Signals/Functions/PS Divide
  PS Product : fl_lib/Physical Signals/Functions/PS Product
      settings: LibrarySourceBlock=|
      | fl_ps_legacy_lib/Legacy Physical
      | Signals/Functions/PS Product
  PS-Simulink Converter1 : nesl_utility/PS-Simulink Converter  PhysicalDomain=network_engine_domain  SubClassName=ps_output  LeftPortType=input  RightPortType=output  PseudoPeriodic=off  Frequencies=[]  VectorFormat=1-D array  Unit=m  AffineConversion=off
  PS-Simulink Converter17 : nesl_utility/PS-Simulink Converter  PhysicalDomain=network_engine_domain  SubClassName=ps_output  LeftPortType=input  RightPortType=output  PseudoPeriodic=off  Frequencies=[]  VectorFormat=1-D array  Unit=N/m  AffineConversion=off
  Scope : Scope
  Scope1 : Scope
  Terminator : Terminator
  SpringRate : PMIOPort  Side=Right
  Pos : PMIOPort  Port=2  Side=Left
  wires:
  PS-Simulink Converter17/1 -> Scope1/1, Terminator/1  "SlideSprRate"
  PS-Simulink Converter1/1 -> Scope/1
  connections:
  E (Pa)/RConn1 -- PS Product/LConn1
  A (m^2)/RConn1 -- PS Product/LConn2
  PS Product/RConn1 -- PS Divide/LConn1
  PS Divide/RConn1 -- PS-Simulink Converter17/LConn1 -- SpringRate/RConn1
  L_initial (m)/RConn1 -- PS Add/LConn1
  PS Divide/LConn2 -- PS-Simulink Converter1/LConn1 -- PS Add/RConn1
  PS Add/LConn2 -- Pos/RConn1

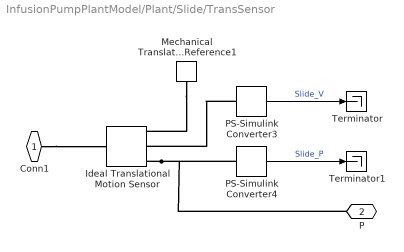
== system InfusionPumpPlantModel/Plant/Slide/TransSensor ==
  Ideal Translational Motion Sensor : fl_lib/Mechanical/Mechanical Sensors/Ideal Translational Motion Sensor  reference=foundation.enum.MeasurementReference.difference  acceleration_port=false  velocity_port=true  position_port=true  offset=0 m
  Mechanical Translational Reference1 : fl_lib/Mechanical/Translational Elements/Mechanical Translational Reference
  PS-Simulink Converter3 : nesl_utility/PS-Simulink Converter  PhysicalDomain=network_engine_domain  SubClassName=ps_output  LeftPortType=input  RightPortType=output  PseudoPeriodic=off  Frequencies=[]  VectorFormat=1-D array  Unit=mm/s  AffineConversion=off
  PS-Simulink Converter4 : nesl_utility/PS-Simulink Converter  PhysicalDomain=network_engine_domain  SubClassName=ps_output  LeftPortType=input  RightPortType=output  PseudoPeriodic=off  Frequencies=[]  VectorFormat=1-D array  Unit=mm  AffineConversion=off
  Terminator : Terminator
  Terminator1 : Terminator
  Conn1 : PMIOPort  Side=Left
  P : PMIOPort  Port=2  Side=Right
  wires:
  PS-Simulink Converter4/1 -> Terminator1/1  "Slide_P"
  PS-Simulink Converter3/1 -> Terminator/1  "Slide_V"
  connections:
  Conn1/RConn1 -- Ideal Translational Motion Sensor/LConn1
  Ideal Translational Motion Sensor/RConn3 -- P/RConn1 -- PS-Simulink Converter4/LConn1
  PS-Simulink Converter3/LConn1 -- Ideal Translational Motion Sensor/RConn2
  Mechanical Translational Reference1/LConn1 -- Ideal Translational Motion Sensor/RConn1
